simulink model "nms_sim_2D_cost"  (R2024b)
settings: Solver=ode15s  StartTime=0.0  StopTime=t_sim  MaxStep=dt_max  EnableMultiTasking=on
values from neighbouring files (symbols this model uses):
  a_BFSH = param_ctrl(35)*1    [setCtrlPar_optim_CPGreflex2001_2D.m]
  a_GAS = param_ctrl(37)*1    [setCtrlPar_optim_CPGreflex2001_2D.m]
  a_GLU = param_ctrl(31)*1    [setCtrlPar_optim_CPGreflex2001_2D.m]
  a_HAM = param_ctrl(33)*1    [setCtrlPar_optim_CPGreflex2001_2D.m]
  a_HFL = param_ctrl(32)*1    [setCtrlPar_optim_CPGreflex2001_2D.m]
  a_RF = param_ctrl(34)*1    [setCtrlPar_optim_CPGreflex2001_2D.m]
  a_SOL = param_ctrl(38)*1    [setCtrlPar_optim_CPGreflex2001_2D.m]
  a_TA = param_ctrl(39)*1    [setCtrlPar_optim_CPGreflex2001_2D.m]
  a_VAS = param_ctrl(36)*1    [setCtrlPar_optim_CPGreflex2001_2D.m]
  ai = param_ctrl(96)*2.0    [setCtrlPar_optim_CPGreflex2001_2D.m]
  b_BFSH = param_ctrl(52)*.51    [setCtrlPar_optim_CPGreflex2001_2D.m]
  b_BFSHGAS = param_ctrl(55)*.51    [setCtrlPar_optim_CPGreflex2001_2D.m]
  b_BFSHHAM = param_ctrl(54)*.51    [setCtrlPar_optim_CPGreflex2001_2D.m]
  b_BFSHVAS = param_ctrl(53)*.51    [setCtrlPar_optim_CPGreflex2001_2D.m]
  b_GAS = param_ctrl(59)*.51    [setCtrlPar_optim_CPGreflex2001_2D.m]
  b_GASBFSH = param_ctrl(60)*.51    [setCtrlPar_optim_CPGreflex2001_2D.m]
  b_GASSOL = param_ctrl(61)*.51    [setCtrlPar_optim_CPGreflex2001_2D.m]
  b_GLU = param_ctrl(40)*.51    [setCtrlPar_optim_CPGreflex2001_2D.m]
  b_GLUHAM = param_ctrl(42)*.51    [setCtrlPar_optim_CPGreflex2001_2D.m]
  b_GLUHFL = param_ctrl(41)*.51    [setCtrlPar_optim_CPGreflex2001_2D.m]
  b_HAM = param_ctrl(46)*.51    [setCtrlPar_optim_CPGreflex2001_2D.m]
  b_HAMBFSH = param_ctrl(48)*.51    [setCtrlPar_optim_CPGreflex2001_2D.m]
  b_HAMGLU = param_ctrl(47)*.51    [setCtrlPar_optim_CPGreflex2001_2D.m]
  b_HFL = param_ctrl(43)*.51    [setCtrlPar_optim_CPGreflex2001_2D.m]
  b_HFLGLU = param_ctrl(44)*.51    [setCtrlPar_optim_CPGreflex2001_2D.m]
  b_HFLRF = param_ctrl(45)*.51    [setCtrlPar_optim_CPGreflex2001_2D.m]
  b_RF = param_ctrl(49)*.51    [setCtrlPar_optim_CPGreflex2001_2D.m]
  b_RFHFL = param_ctrl(50)*.51    [setCtrlPar_optim_CPGreflex2001_2D.m]
  b_RFVAS = param_ctrl(51)*.51    [setCtrlPar_optim_CPGreflex2001_2D.m]
  b_SOL = param_ctrl(62)*.51    [setCtrlPar_optim_CPGreflex2001_2D.m]
  b_SOLGAS = param_ctrl(64)*.51    [setCtrlPar_optim_CPGreflex2001_2D.m]
  b_SOLTA = param_ctrl(63)*.51    [setCtrlPar_optim_CPGreflex2001_2D.m]
  b_TA = param_ctrl(65)*.51    [setCtrlPar_optim_CPGreflex2001_2D.m]
  b_TASOL = param_ctrl(66)*.51    [setCtrlPar_optim_CPGreflex2001_2D.m]
  b_VAS = param_ctrl(56)*.51    [setCtrlPar_optim_CPGreflex2001_2D.m]
  b_VASBFSH = param_ctrl(57)*.51    [setCtrlPar_optim_CPGreflex2001_2D.m]
  b_VASRF = param_ctrl(58)*.51    [setCtrlPar_optim_CPGreflex2001_2D.m]
  bias = param_ctrl(97)*2.5    [setCtrlPar_optim_CPGreflex2001_2D.m]
  c = 0.05    [nms_MS_2D_scaled.m]
  c_jointstop = 0.3 / (pi/180)    (= 17.1887338539)    [nms_MS_2D_scaled.m]
  D12_F = 0.16    *scaleL_JPhys    [nms_MechInit_2D_scaleSkel.m]
  D12_S = 0.2460	*sub_height    [nms_MechInit_2D_scaleSkel.m]
  D12_T = 0.2450  *sub_height    [nms_MechInit_2D_scaleSkel.m]
  D12y_F = 0.039  *sub_height    [nms_MechInit_2D_scaleSkel.m]
  D12z_HAT = 0.1    [nms_MS_2D_scaled.m]
  D13_F = 0.20    *scaleL_JPhys    [nms_MechInit_2D_scaleSkel.m]
  D1G_F = 0.14    *scaleL_JPhys    [nms_MechInit_2D_scaleSkel.m]
  D1G_HAT = 0.35  *scaleL_JPhys    [nms_MechInit_2D_scaleSkel.m]
  D1G_S = (0.3 - D12y_F/4)	*scaleL_JPhys    [nms_MechInit_2D_scaleSkel.m]
  D1G_T = (0.3 - D12y_F/4)	*scaleL_JPhys    [nms_MechInit_2D_scaleSkel.m]
  D1Gy_F = D12y_F*D1G_F/D12_F    (= 0.07)    [nms_MechInit_2D_scaleSkel.m]
  d_BFSH = param_ctrl(26)*1    [setCtrlPar_optim_CPGreflex2001_2D.m]
  d_GAS = param_ctrl(28)*1    [setCtrlPar_optim_CPGreflex2001_2D.m]
  d_GLU = param_ctrl(22)*1    [setCtrlPar_optim_CPGreflex2001_2D.m]
  d_HAM = param_ctrl(24)*1    [setCtrlPar_optim_CPGreflex2001_2D.m]
  d_HFL = param_ctrl(23)*1    [setCtrlPar_optim_CPGreflex2001_2D.m]
  d_RF = param_ctrl(25)*1    [setCtrlPar_optim_CPGreflex2001_2D.m]
  d_SOL = param_ctrl(29)*1    [setCtrlPar_optim_CPGreflex2001_2D.m]
  d_TA = param_ctrl(30)*1    [setCtrlPar_optim_CPGreflex2001_2D.m]
  d_VAS = param_ctrl(27)*1    [setCtrlPar_optim_CPGreflex2001_2D.m]
  DeltaThRef = 5e-3    (= 0.005)    [nms_MS_2D_scaled.m]
  dloptBFSH = 3.0    (= 3)    [setCtrlPar_optim_CPGreflex2001_2D.m]
  dloptGAS = 3.0    (= 3)    [setCtrlPar_optim_CPGreflex2001_2D.m]
  dloptGLU = 3.0    (= 3)    [setCtrlPar_optim_CPGreflex2001_2D.m]
  dloptHAM = 3.0    (= 3)    [setCtrlPar_optim_CPGreflex2001_2D.m]
  dloptHFL = 3.0    (= 3)    [setCtrlPar_optim_CPGreflex2001_2D.m]
  dloptRF = 3.0    (= 3)    [setCtrlPar_optim_CPGreflex2001_2D.m]
  dloptSOL = 3.0    (= 3)    [setCtrlPar_optim_CPGreflex2001_2D.m]
  dloptTA = 3.0    (= 3)    [setCtrlPar_optim_CPGreflex2001_2D.m]
  dloptVAS = 3.0    (= 3)    [setCtrlPar_optim_CPGreflex2001_2D.m]
  ec_BFSH = param_ctrl(80)*0.15    [setCtrlPar_optim_CPGreflex2001_2D.m]
  ec_GAS = param_ctrl(82)*0.15    [setCtrlPar_optim_CPGreflex2001_2D.m]
  ec_GLU = param_ctrl(76)*0.15    [setCtrlPar_optim_CPGreflex2001_2D.m]
  ec_HAM = param_ctrl(78)*0.15    [setCtrlPar_optim_CPGreflex2001_2D.m]
  ec_HFL = param_ctrl(77)*0.15    [setCtrlPar_optim_CPGreflex2001_2D.m]
  ec_RF = param_ctrl(79)*0.15    [setCtrlPar_optim_CPGreflex2001_2D.m]
  ec_TA = param_ctrl(84)*0.15    [setCtrlPar_optim_CPGreflex2001_2D.m]
  ec_VAS = param_ctrl(81)*0.15    [setCtrlPar_optim_CPGreflex2001_2D.m]
  eref = 0.04    [nms_MS_2D_scaled.m]
  eref_GAS = 0.1    [nms_MS_2D_scaled.m]
  eref_SOL = 0.1    [nms_MS_2D_scaled.m]
  es_BFSH = param_ctrl(89)*0.15    [setCtrlPar_optim_CPGreflex2001_2D.m]
  es_GAS = param_ctrl(91)*0.15    [setCtrlPar_optim_CPGreflex2001_2D.m]
  es_GLU = param_ctrl(85)*0.15    [setCtrlPar_optim_CPGreflex2001_2D.m]
  es_HAM = param_ctrl(87)*0.15    [setCtrlPar_optim_CPGreflex2001_2D.m]
  es_HFL = param_ctrl(86)*0.15    [setCtrlPar_optim_CPGreflex2001_2D.m]
  es_RF = param_ctrl(88)*0.15    [setCtrlPar_optim_CPGreflex2001_2D.m]
  es_TA = param_ctrl(93)*0.15    [setCtrlPar_optim_CPGreflex2001_2D.m]
  es_VAS = param_ctrl(90)*0.15    [setCtrlPar_optim_CPGreflex2001_2D.m]
  FmaxBFSH = 350    [nms_MS_2D_scaled.m]
  FmaxGAS = 2000    [nms_MS_2D_scaled.m]
  FmaxGLU = 4000    [nms_MS_2D_scaled.m]
  FmaxHAM = 2000    [nms_MS_2D_scaled.m]
  FmaxHFL = 2000    [nms_MS_2D_scaled.m]
  FmaxRF = 850    [nms_MS_2D_scaled.m]
  FmaxSOL = 4000    [nms_MS_2D_scaled.m]
  FmaxTA = 800    [nms_MS_2D_scaled.m]
  FmaxVAS = 5000    [nms_MS_2D_scaled.m]
  g = 9.81    [nms_MS_2D_scaled.m]
  gamma_4 = param_ctrl(11) * 1.7    [setCtrlPar_optim_CPGreflexsynergy2023_2D.m]
  h_BFSH = param_ctrl(71)*.1    [setCtrlPar_optim_CPGreflex2001_2D.m]
  h_GAS = param_ctrl(73)*.1    [setCtrlPar_optim_CPGreflex2001_2D.m]
  h_GLU = param_ctrl(67)*.1    [setCtrlPar_optim_CPGreflex2001_2D.m]
  h_HAM = param_ctrl(69)*.1    [setCtrlPar_optim_CPGreflex2001_2D.m]
  h_HFL = param_ctrl(68)*.1    [setCtrlPar_optim_CPGreflex2001_2D.m]
  h_RF = param_ctrl(70)*.1    [setCtrlPar_optim_CPGreflex2001_2D.m]
  h_SOL = param_ctrl(74)*.1    [setCtrlPar_optim_CPGreflex2001_2D.m]
  h_TA = param_ctrl(75)*.1    [setCtrlPar_optim_CPGreflex2001_2D.m]
  h_VAS = param_ctrl(72)*.1    [setCtrlPar_optim_CPGreflex2001_2D.m]
  HLCtrlPar = [theta_tgt l_clr alpha_tgt alpha_cd alpha_cv]    [setCtrlPar_optim_reflex2015_2D.m]
  In_F = 0.005    *scaleM*scaleL_JPhys^2    [nms_MechInit_2D_scaleSkel.m]
  In_HAT = 2.5    *scaleM*scaleL_JPhys^2    [nms_MechInit_2D_scaleSkel.m]
  In_S = 0.05     *scaleM*scaleL_JPhys^2    [nms_MechInit_2D_scaleSkel.m]
  In_T = 0.15     *scaleM*scaleL_JPhys^2    [nms_MechInit_2D_scaleSkel.m]
  init_exc = 0.01    [setInitPar_optim_2D.m]
  init_fm = 0.01    [setInitPar_optim_2D.m]
  init_lce = 1    [setInitPar_optim_2D.m]
  init_LCPG = param_ctrl(12) * 0.01    [setCtrlPar_optim_CPGreflexsynergy2023_2D.m]
  init_LStance = 1    [setInitPar_optim_2D.m]
  init_N1 = osc_signal1(phi_off_osc_ind)    [setCtrlPar_optim_CPGreflex2001_2D.m]
  ... (+441 more)
undefined symbols (not defined in the file or in its folder): cost_act_exponent, cost_v_tgt, flag_controller, Newton, nStep_obj, nStep_startKin, Raphson, sgn, SSW_kin, terrain_slope_angle, v_plateS1, X, Y, Z
libraries: nesl_utility x94, sm_lib x90, simulink x28, simulink_extras x12
(part 18 of 20)

== system nms_sim_2D_cost/Muscle synergy Controller/Right Movement Regulator/Right Trunk Balance ==
  note: GLU
  note: HFL
  theta : Inport
  dtheta : Inport  Port=2
  RStance : EnablePort  StatesWhenEnabling=reset
  Constant : Constant  Value=theta_trunk_tgt
  Constant1 : Constant  Value=k_HFL
  Constant2 : Constant  Value=sigma_HFL
  Constant3 : Constant  Value=theta_trunk_tgt
  Constant4 : Constant  Value=k_GLU
  Constant5 : Constant  Value=sigma_GLU
  Gain : Gain  Gain=-1
  Gain1 : Gain  Gain=-1
  Product{,1..3} (4 alike) : Product
  Sum{,1..3} (4 alike) : Sum  Inputs=|+-
  RExcHFL_MR : Outport  OutputWhenDisabled=reset  InitialOutput=0
  RExcGLU_MR : Outport  Port=2
  wires:
  dtheta/1 -> Product1/2, Product3/2
  Constant3/1 -> Sum2/2
  Constant4/1 -> Gain1/1
  theta/1 -> Sum/1, Sum2/1
  Sum2/1 -> Product2/1  "theta - theta_tgt"
  Gain1/1 -> Product2/2  "-K_GLU"
  Product3/1 -> Sum3/2
  Sum3/1 -> RExcGLU_MR/1
  Product2/1 -> Sum3/1
  Constant5/1 -> Product3/1
  Sum/1 -> Product/1  "theta - theta_tgt"
  Product1/1 -> Sum1/2
  Product/1 -> Sum1/1
  Constant/1 -> Sum/2
  Gain/1 -> Product/2  "-K_HFL"
  Constant2/1 -> Product1/1
  Constant1/1 -> Gain/1
  Sum1/1 -> RExcHFL_MR/1

== system nms_sim_2D_cost/Reflex Controller/Higher Control Layer (Supraspinal Control)/Stance to Swing ==
  LStance : Inport
  RStance : Inport  Port=2
  Lalpha_tgt : Inport  Port=3
  Lphi34 : Inport  Port=4
  Lphi23 : Inport  Port=5
  Ralpha_tgt : Inport  Port=6
  Rphi34 : Inport  Port=7
  Rphi23 : Inport  Port=8
  Abs : Abs  ZeroCross=off  SaturateOnIntegerOverflow=off
  Abs1 : Abs  ZeroCross=off  SaturateOnIntegerOverflow=off
  Lalpha' : Fcn  Expr=u(1) - u(2)/2
  Logical Operator1 : Logic  Operator=NOR  AllPortsSameDT=off  OutDataTypeStr=boolean
  Logical Operator2 : Logic  Operator=NOT  AllPortsSameDT=off
  Logical Operator3 : Logic  AllPortsSameDT=off
  Logical Operator4 : Logic  AllPortsSameDT=off
  Logical Operator5 : Logic  AllPortsSameDT=off
  Mux1 : Mux  Inputs=2
  Mux5 : Mux  Inputs=2
  Ralpha' : Fcn  Expr=u(1) - u(2)/2
  Relational Operator : RelationalOperator  Operator=>  ZeroCross=off  InputSameDT=off
  Sum5 : Sum  Inputs=-+|
  Sum7 : Sum  Inputs=-+|
  LSwInit : Outport  VectorParamsAs1DForOutWhenUnconnected=off
  Flight : Outport  Port=2  VectorParamsAs1DForOutWhenUnconnected=off
  RSwInit : Outport  Port=3  VectorParamsAs1DForOutWhenUnconnected=off
  wires:
  Lalpha'/1 -> Sum7/2  "Lalpha"
  Mux5/1 -> Lalpha'/1
  Ralpha'/1 -> Sum5/2
  Mux1/1 -> Ralpha'/1
  Sum5/1 -> Abs/1
  Sum7/1 -> Abs1/1
  Abs1/1 -> Relational Operator/1
  Abs/1 -> Relational Operator/2
  Logical Operator3/1 -> Logical Operator4/1, Logical Operator5/1
  LStance/1 -> Logical Operator3/1, Logical Operator1/1
  RStance/1 -> Logical Operator3/2, Logical Operator1/2
  Lalpha_tgt/1 -> Sum7/1
  Lphi34/1 -> Mux5/1
  Lphi23/1 -> Mux5/2
  Ralpha_tgt/1 -> Sum5/1
  Rphi34/1 -> Mux1/1
  Rphi23/1 -> Mux1/2
  Logical Operator1/1 -> Flight/1
  Relational Operator/1 -> Logical Operator2/1, Logical Operator4/2
  Logical Operator4/1 -> LSwInit/1
  Logical Operator2/1 -> Logical Operator5/2
  Logical Operator5/1 -> RSwInit/1

== system nms_sim_2D_cost/Reflex Controller/Lower Control Layer (Spinal Cord)/L Stance Phase ==
  note: Left Stance Phase Control
  note: M1: realize compliant leg
  note: M2: prevent knee overextension
  note: M3: balance trunk
  note: 0: Pre-excitations
  note: M5: flex ankle
  note: M4: compensate swing leg
  CtrlPar : Inport
  theta_tgt [rad] : Inport  Port=2
  theta dtheta [rad rad/s] : Inport  Port=3
  CExc_HSw : Inport  Port=4
  FmGLU : Inport  Port=5
  FmHAM : Inport  Port=6
  FmVAS : Inport  Port=7
  LceBFSH : Inport  Port=8
  FmGAS : Inport  Port=9
  FmSOL : Inport  Port=10
  LceTA : Inport  Port=11
  Enable : EnablePort  StatesWhenEnabling=reset  ZeroCross=off
  Demux1 : Demux  Outputs=5
  Demux3 : Demux  Outputs=3
  Demux4 : Demux
  Demux5 : Demux  Outputs=5
  Demux6 : Demux  Outputs=3
  Demux7 : Demux  Outputs=2
  Demux8 : Demux  Outputs=6
  Divide{4..17,19..22,25} (19 alike) : Product
  Gain : Gain  Gain=-1
  Gain2 : Gain  Gain=-1
  Gain3 : Gain  Gain=-1
  Mux{1..3,5} (4 alike) : Mux  Inputs=3
  Mux4 : Mux
  Sum{1,3..5} (4 alike) : Sum  Inputs=-+|  InputSameDT=on  SaturateOnIntegerOverflow=on  OutDataTypeStr=Inherit: Same as first input
  Sum{2,7..8,11} (4 alike) : Sum  Inputs=|++  InputSameDT=on  SaturateOnIntegerOverflow=on  OutDataTypeStr=Inherit: Same as first input
  Sum6 : Sum  Inputs=+-|  InputSameDT=on  SaturateOnIntegerOverflow=on  OutDataTypeStr=Inherit: Same as first input
  parStPreE : Selector  InputPortWidth=St_i  IndexOptions=Index vector (dialog)  Indices=parSt_PreE_i  OutputSizes=1
  parSt_M1 : Selector  InputPortWidth=St_i  IndexOptions=Index vector (dialog)  Indices=parSt_M1_i  OutputSizes=1
  parSt_M2 : Selector  InputPortWidth=St_i  IndexOptions=Index vector (dialog)  Indices=parSt_M2_i  OutputSizes=1
  parSt_M3 : Selector  InputPortWidth=St_i  IndexOptions=Index vector (dialog)  Indices=parSt_M3_i  OutputSizes=1
  parSt_M4 : Selector  InputPortWidth=St_i  IndexOptions=Index vector (dialog)  Indices=parSt_M4_i  OutputSizes=1
  parSt_M5 : Selector  InputPortWidth=St_i  IndexOptions=Index vector (dialog)  Indices=parSt_M5_i  OutputSizes=1
  positive half{1..6} (6 alike) : Saturate  UpperLimit=inf  LowerLimit=0  ZeroCross=off
  E_St_0 : Outport  OutputWhenDisabled=reset  InitialOutput=0  VectorParamsAs1DForOutWhenUnconnected=off
  E_M1 [GLU VAS SOL] : Outport  Port=2  OutputWhenDisabled=reset  InitialOutput=0  VectorParamsAs1DForOutWhenUnconnected=off
  E_M2 [HAM VAS BFSH GAS] : Outport  Port=3  OutputWhenDisabled=reset  InitialOutput=0  VectorParamsAs1DForOutWhenUnconnected=off
  E_M3 [HFL GLU HAM] : Outport  Port=4  OutputWhenDisabled=reset  InitialOutput=0  VectorParamsAs1DForOutWhenUnconnected=off
  E_M4 [HFL GLU HAM] : Outport  Port=5  OutputWhenDisabled=reset  InitialOutput=0  VectorParamsAs1DForOutWhenUnconnected=off
  E_M5 [TA] : Outport  Port=6  OutputWhenDisabled=reset  InitialOutput=0  VectorParamsAs1DForOutWhenUnconnected=off
  wires:
  Demux5/2 -> Divide20/2  "GainDTh_HFL"
  Divide11/1 -> Mux4/4  "GAS"
  Divide15/1 -> Gain/1
  Divide13/1 -> Mux4/3  "BFSH"
  Mux2/1 -> E_M1 [GLU VAS SOL]/1
  positive half3/1 -> Divide15/1
  Demux8/2 -> Sum3/1  "loff_BFSH_VAS"
  Demux8/6 -> Divide11/1  "FGain_GAS"
  Demux8/5 -> Divide13/2  "LGain_BFSH"
  Sum3/1 -> positive half3/1
  Divide7/1 -> Mux2/1  "GLU"
  LceBFSH/1 -> Sum3/2, Sum4/2
  Demux5/1 -> Divide19/2  "GainTh_HFL"
  FmGLU/1 -> Divide7/2
  parSt_M1/1 -> Demux3/1
  positive half6/1 -> Mux1/3
  Demux7/2 -> Gain3/1, Divide5/1  "dtheta"
  Sum2/1 -> positive half1/1  "HFL"
  Sum4/1 -> positive half4/1
  Divide10/1 -> Mux2/3  "SOL"
  positive half2/1 -> Mux1/2
  Divide14/1 -> Mux4/1  "HAM"
  theta_tgt [rad]/1 -> Sum1/1
  Demux5/5 -> Divide6/2  "SGainGLU_HAM"
  Divide6/1 -> positive half6/1  "HAM"
  positive half1/1 -> Mux1/1
  Mux1/1 -> E_M3 [HFL GLU HAM]/1
  Divide5/1 -> Sum8/2
  Demux8/3 -> Divide15/2  "LGainBFSH_VAS"
  parSt_M2/1 -> Demux8/1
  Demux8/1 -> Divide14/1  "FGain_HAM"
  Gain/1 -> Mux4/2  "VAS"
  Sum8/1 -> Divide6/1, positive half2/1  "GLU"
  Demux5/3 -> Divide4/2  "GainTh_GLU"
  Gain2/1 -> Divide19/1
  Divide20/1 -> Sum2/2
  Gain3/1 -> Divide20/1
  Divide19/1 -> Sum2/1
  parSt_M3/1 -> Demux5/1
  Divide4/1 -> Sum8/1
  Demux3/3 -> Divide10/1  "FGain_SOL"
  FmHAM/1 -> Divide14/2
  theta dtheta [rad rad/s]/1 -> Demux7/1
  Sum1/1 -> Gain2/1, Divide4/1
  Demux7/1 -> Sum1/2  "theta"
  Demux5/4 -> Divide5/2  "GainDTh_GLU"
  FmGAS/1 -> Divide11/2
  Demux8/4 -> Sum4/1  "loff_BFSH"
  FmVAS/1 -> Divide8/2
  Demux3/1 -> Divide7/1  "FGain_GLU"
  positive half4/1 -> Divide13/1
  Divide8/1 -> Mux2/2  "VAS"
  Demux3/2 -> Divide8/1  "FGain_VAS"
  Mux4/1 -> E_M2 [HAM VAS BFSH GAS]/1
  parStPreE/1 -> E_St_0/1
  Sum6/1 -> E_M5 [TA]/1  "TA"
  Demux1/5 -> Divide21/2  "SGainGLU_HAM"
  Divide12/1 -> Sum11/1
  Sum11/1 -> Mux5/2, Divide21/1  "GLU"
  Demux4/4 -> Divide9/2  "Exc_CRF"
  Divide21/1 -> Mux5/3  "HAM"
  CExc_HSw/1 -> Demux4/1
  Demux1/4 -> Divide9/1  "SGainCRF_GLU"
  Divide17/1 -> Sum7/2
  Demux1/2 -> Divide17/1  "SGainCHAM_HFL"
  Demux4/2 -> Divide22/2  "Exc_CGLU"
  Sum7/1 -> Mux5/1  "HFL"
  positive half5/1 -> Divide16/1
  Demux1/1 -> Divide22/1  "SGainCGLU_HFL"
  Demux4/1 -> Divide12/2  "Exc_CHFL"
  Demux4/3 -> Divide17/2  "Exc_CHAM"
  Divide9/1 -> Sum11/2
  Demux1/3 -> Divide12/1  "SGainCHFL_GLU"
  parSt_M4/1 -> Demux1/1
  Demux6/3 -> Divide25/2  "FGainSOL_TA"
  Demux6/1 -> Sum5/1  "loffTA"
  Demux6/2 -> Divide16/2  "LGain_TA"
  CtrlPar/1 -> parStPreE/1, parSt_M1/1, parSt_M2/1, parSt_M5/1, parSt_M4/1, parSt_M3/1
  Divide25/1 -> Sum6/2
  Mux5/1 -> E_M4 [HFL GLU HAM]/1
  Divide22/1 -> Sum7/1
  Sum5/1 -> positive half5/1
  Divide16/1 -> Sum6/1
  parSt_M5/1 -> Demux6/1
  FmSOL/1 -> Divide25/1, Divide10/2
  LceTA/1 -> Sum5/2

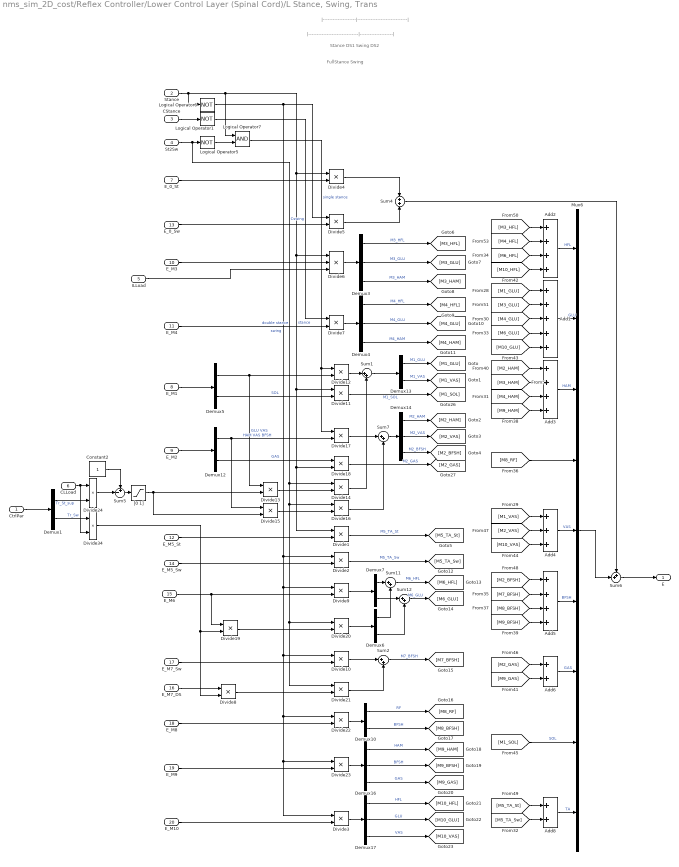
== system nms_sim_2D_cost/Reflex Controller/Lower Control Layer (Spinal Cord)/L Stance, Swing, Trans ==
  note: Stance DS1 Swing DS2
  note: FullStance Swing
  note: |------------------------------|--------------------|
  note: |--------------------|------------------------------|
  CtrlPar : Inport
  Stance : Inport  Port=2
  CStance : Inport  Port=3
  St2Sw : Inport  Port=4
  ILLoad : Inport  Port=5
  CLLoad : Inport  Port=6
  E_0_St : Inport  Port=7
  E_M1 : Inport  Port=8
  E_M2 : Inport  Port=9
  E_M3 : Inport  Port=10
  E_M4 : Inport  Port=11
  E_M5_St : Inport  Port=12
  E_0_Sw : Inport  Port=13
  E_M5_Sw : Inport  Port=14
  E_M6 : Inport  Port=15
  E_M7_DS : Inport  Port=16
  E_M7_Sw : Inport  Port=17
  E_M8 : Inport  Port=18
  E_M9 : Inport  Port=19
  E_M10 : Inport  Port=20
  Add1 : Sum  Inputs=5
  Add2 : Sum  Inputs=4
  Add3 : Sum  Inputs=4
  Add4 : Sum  Inputs=3
  Add5 : Sum  Inputs=4
  Add6 : Sum  Inputs=2
  Add8 : Sum  Inputs=2
  Constant2 : Constant
  Demux{1,6..7,10,13} (5 alike) : Demux  Outputs=2
  Demux12 : Demux  Outputs=[3 1]
  Demux{3..4,14,16..17} (5 alike) : Demux  Outputs=3
  Demux5 : Demux  Outputs=[2 1]
  Divide{1..5,7..24,34} (24 alike) : Product
  Divide6 : Product  Inputs=3
  Logical Operator1 : Logic  Operator=NOT  AllPortsSameDT=off  OutDataTypeStr=boolean
  Logical Operator5 : Logic  Operator=NOT  AllPortsSameDT=off  OutDataTypeStr=boolean
  Logical Operator6 : Logic  Operator=NOT  AllPortsSameDT=off  OutDataTypeStr=boolean
  Logical Operator7 : Logic  AllPortsSameDT=off  OutDataTypeStr=boolean
  Mux6 : Mux  Inputs=9
  Sum{1..2,7,11..12} (5 alike) : Sum  Inputs=|++  InputSameDT=on  SaturateOnIntegerOverflow=on  OutDataTypeStr=Inherit: Same as first input
  Sum4 : Sum  InputSameDT=on  SaturateOnIntegerOverflow=on  OutDataTypeStr=Inherit: Same as first input
  Sum5 : Sum  Inputs=+-|  InputSameDT=on  SaturateOnIntegerOverflow=on  OutDataTypeStr=Inherit: Same as first input
  Sum6 : Sum  Inputs=++|  InputSameDT=on  SaturateOnIntegerOverflow=on  OutDataTypeStr=Inherit: Same as first input
  "[0 1]" : Saturate  UpperLimit=1  LowerLimit=0  ZeroCross=off
  E : Outport  OutputWhenDisabled=reset  InitialOutput=0  VectorParamsAs1DForOutWhenUnconnected=off
  wires:
  CtrlPar/1 -> Demux1/1
  Stance/1 -> Logical Operator6/1, Logical Operator7/1, Divide4/1, Divide11/1, Divide18/2, Divide1/1, Divide6/1  "stance"
  St2Sw/1 -> Logical Operator5/1, Divide14/1, Divide16/1, Divide20/1, Divide21/1  "double stance"
  Logical Operator5/1 -> Logical Operator7/2
  E_M4/1 -> Divide7/2
  CStance/1 -> Logical Operator1/1
  Logical Operator1/1 -> Divide7/1  "Cswing"
  Demux1/1 -> Divide24/2  "Tr_St_sup"
  Divide24/1 -> Sum5/2
  Constant2/1 -> Sum5/1
  CLLoad/1 -> Divide24/1, Divide34/2
  Demux4/1 -> [M4_HFL]  "M4_HFL"
  Add2/1 -> Mux6/1  "HFL"
  Add1/1 -> Mux6/2  "GLU"
  Demux4/2 -> [M4_GLU]  "M4_GLU"
  Add3/1 -> Mux6/3  "HAM"
  Demux4/3 -> [M4_HAM]  "M4_HAM"
  Add4/1 -> Mux6/5  "VAS"
  Add5/1 -> Mux6/6  "BFSH"
  Add6/1 -> Mux6/7  "GAS"
  Add8/1 -> Mux6/9  "TA"
  Demux1/2 -> Divide34/1  "Tr_Sw"
  Divide7/1 -> Demux4/1
  Logical Operator7/1 -> Divide12/1, Divide17/1  "single stance"
  Divide34/1 -> Divide19/2, Divide8/2
  Logical Operator6/1 -> Divide5/1, Divide2/1, Divide9/1, Divide10/1, Divide23/1, Divide3/1, Divide22/1  "swing"
  Mux6/1 -> Sum6/2
  Sum6/1 -> E/1
  Sum4/1 -> Sum6/1
  E_0_Sw/1 -> Divide5/2
  E_0_St/1 -> Divide4/2
  Divide5/1 -> Sum4/2
  Divide4/1 -> Sum4/1
  E_M1/1 -> Demux5/1
  E_M2/1 -> Demux12/1
  Demux5/1 -> Divide12/2, Divide13/1  "GLU VAS"
  Demux5/2 -> Divide11/2  "SOL"
  Divide12/1 -> Sum1/1
  Divide13/1 -> Divide14/2
  Divide14/1 -> Sum1/2
  Divide16/1 -> Sum7/2
  Divide15/1 -> Divide16/2
  Sum1/1 -> Demux13/1
  Demux13/1 -> [M1_GLU]  "M1_GLU"
  Demux13/2 -> [M1_VAS]  "M1_VAS"
  Demux12/1 -> Divide17/2, Divide15/1  "HAM VAS BFSH"
  Divide17/1 -> Sum7/1
  Sum7/1 -> Demux14/1
  Demux14/1 -> [M2_HAM]  "M2_HAM"
  Demux14/2 -> [M2_VAS]  "M2_VAS"
  Demux14/3 -> [M2_BFSH]  "M2_BFSH"
  Demux12/2 -> Divide18/1  "GAS"
  Divide18/1 -> [M2_GAS]  "M2_GAS"
  E_M5_St/1 -> Divide1/2
  Divide1/1 -> [M5_TA_St]  "M5_TA_St"
  Divide11/1 -> [M1_SOL]  "M1_SOL"
  E_M3/1 -> Divide6/2
  ILLoad/1 -> Divide6/3
  Divide6/1 -> Demux3/1
  Demux3/1 -> [M3_HFL]  "M3_HFL"
  Demux3/2 -> [M3_GLU]  "M3_GLU"
  Demux3/3 -> [M3_HAM]  "M3_HAM"
  E_M5_Sw/1 -> Divide2/2
  Divide2/1 -> [M5_TA_Sw]  "M5_TA_Sw"
  E_M6/1 -> Divide9/2, Divide19/1
  Divide9/1 -> Demux7/1
  Demux7/2 -> Sum12/1
  Divide20/1 -> Demux6/1
  Demux6/1 -> Sum11/2
  Demux6/2 -> Sum12/2
  Demux7/1 -> Sum11/1
  Divide19/1 -> Divide20/2
  Sum11/1 -> [M6_HFL]  "M6_HFL"
  Sum12/1 -> [M6_GLU]  "M6_GLU"
  Divide10/1 -> Sum2/1
  Divide21/1 -> Sum2/2
  Sum5/1 -> "[0 1]"/1
  E_M7_Sw/1 -> Divide10/2
  Divide8/1 -> Divide21/2
  E_M7_DS/1 -> Divide8/1
  Sum2/1 -> [M7_BFSH]  "M7_BFSH"
  E_M8/1 -> Divide22/2
  Divide22/1 -> Demux10/1
  E_M9/1 -> Divide23/2
  Divide23/1 -> Demux16/1
  E_M10/1 -> Divide3/2
  Divide3/1 -> Demux17/1
  Demux10/2 -> [M8_BFSH]  "BFSH"
  Demux10/1 -> [M8_RF]  "RF"
  Demux16/1 -> [M9_HAM]  "HAM"
  Demux16/2 -> [M9_BFSH]  "BFSH"
  Demux16/3 -> [M9_GAS]  "GAS"
  Demux17/1 -> [M10_HFL]  "HFL"
  Demux17/2 -> [M10_GLU]  "GLU"
  Demux17/3 -> [M10_VAS]  "VAS"
  [M1_GLU] -> Add1/1
  [M3_GLU] -> Add1/2
  [M4_GLU] -> Add1/3
  [M6_GLU] -> Add1/4
  [M10_GLU] -> Add1/5
  [M1_VAS] -> Add4/1
  [M2_HAM] -> Add3/1
  [M2_VAS] -> Add4/2
  [M2_BFSH] -> Add5/1
  [M2_GAS] -> Add6/1
  [M3_HFL] -> Add2/1
  [M3_HAM] -> Add3/2
  [M4_HFL] -> Add2/2
  [M4_HAM] -> Add3/3
  [M5_TA_St] -> Add8/1
  [M5_TA_Sw] -> Add8/2
  [M6_HFL] -> Add2/3
  [M7_BFSH] -> Add5/2
  [M9_BFSH] -> Add5/4
  [M8_BFSH] -> Add5/3
  [M8_RF] -> Mux6/4
  [M9_HAM] -> Add3/4
  [M9_GAS] -> Add6/2
  [M10_HFL] -> Add2/4
  [M10_VAS] -> Add4/3
  [M1_SOL] -> Mux6/8  "SOL"
  "[0 1]"/1 -> Divide15/2, Divide13/2

== system nms_sim_2D_cost/Reflex Controller/Lower Control Layer (Spinal Cord)/L Swing Phase ==
  note: Left Swing Phase Control
  note: 0: Pre-excitations
  note: M6: swing hip
  note: M7: flex knee
  note: M8: hold knee
  note: M9: stop leg
  note: M10: prepare stance
  note: M5: flex ankle
  CtrlPar : Inport
  Stance : Inport  Port=2
  a_tgt : Inport  Port=3
  l_clr : Inport  Port=4
  LceRF : Inport  Port=5
  VceRF : Inport  Port=6
  LceHAM : Inport  Port=7
  VceHAM : Inport  Port=8
  lceBFSH : Inport  Port=9
  VceVAS : Inport  Port=10
  VceBFSH : Inport  Port=11
  LceHFL : Inport  Port=12
  LceGLU : Inport  Port=13
  LceVAS : Inport  Port=14
  LceTA : Inport  Port=15
  Enable : EnablePort  StatesWhenEnabling=reset  ZeroCross=off
  Constant1 : Constant  Value=0  OutDataTypeStr=boolean
  Constant10 : Constant  Value=leg_l
  Constant2 : Constant
  Constant3 : Constant
  Constant5 : Constant
  Demux1 : Demux  Outputs=2
  Demux2 : Demux  Outputs=2
  Demux4 : Demux  Outputs=9
  Divide{1..8,22} (9 alike) : Product
  Gain1 : Gain  Gain=-1
  Logical Operator : Logic  Operator=NOT  AllPortsSameDT=off  OutDataTypeStr=boolean
  Logical Operator1 : Logic  AllPortsSameDT=off  OutDataTypeStr=boolean
  Logical Operator2 : Logic  Operator=NOT  AllPortsSameDT=off  OutDataTypeStr=boolean
  Mux1 : Mux  Inputs=3
  Mux2 : Mux  Inputs=2
  Mux3 : Mux  Inputs=2
  Mux4 : Mux  Inputs=3
  Mux8 : Mux  Inputs=2
  Relational Operator : RelationalOperator  Operator=<=  OutDataTypeStr=boolean  ZeroCross=off  InputSameDT=off
  S-R Flip-Flop : simulink_extras/Flip Flops/S-R Flip-Flop  initial_condition=0
  Sum1 : Sum  Inputs=-+|  InputSameDT=on  SaturateOnIntegerOverflow=on  OutDataTypeStr=Inherit: Same as first input
  Sum10 : Sum  Inputs=++|  InputSameDT=on  SaturateOnIntegerOverflow=on  OutDataTypeStr=Inherit: Same as first input
  Sum13 : Sum  Inputs=|+-  InputSameDT=on  SaturateOnIntegerOverflow=on  OutDataTypeStr=Inherit: Same as first input
  Sum14 : Sum  Inputs=|+-  InputSameDT=on  SaturateOnIntegerOverflow=on  OutDataTypeStr=Inherit: Same as first input
  Sum2 : Sum  Inputs=++|  InputSameDT=on  SaturateOnIntegerOverflow=on  OutDataTypeStr=Inherit: Same as first input
  Sum3 : Sum  Inputs=-+|  InputSameDT=on  SaturateOnIntegerOverflow=on  OutDataTypeStr=Inherit: Same as first input
  Sum4 : Sum  Inputs=|+-  InputSameDT=on  SaturateOnIntegerOverflow=on  OutDataTypeStr=Inherit: Same as first input
  Sum5 : Sum  Inputs=+-|  InputSameDT=on  SaturateOnIntegerOverflow=on  OutDataTypeStr=Inherit: Same as first input
  Sum6 : Sum  Inputs=|++  InputSameDT=on  SaturateOnIntegerOverflow=on  OutDataTypeStr=Inherit: Same as first input
  Sum7 : Sum  Inputs=|++  InputSameDT=on  SaturateOnIntegerOverflow=on  OutDataTypeStr=Inherit: Same as first input
  Sum8 : Sum  Inputs=++|  InputSameDT=on  SaturateOnIntegerOverflow=on  OutDataTypeStr=Inherit: Same as first input
  Sum9 : Sum  Inputs=+-|  InputSameDT=on  SaturateOnIntegerOverflow=on  OutDataTypeStr=Inherit: Same as first input
  Terminator : Terminator
  kneei_flexion from alpha : Subsystem  TreatAsAtomicUnit=on
  kneeii_damp and hold & kneeiii_leg stop & kneeiv_stance preparation : Subsystem  TreatAsAtomicUnit=on
  negative half : Saturate  UpperLimit=0  LowerLimit=-inf  ZeroCross=off
  negative half1 : Saturate  UpperLimit=0  LowerLimit=-inf  ZeroCross=off
  negative half2 : Saturate  UpperLimit=0  LowerLimit=-inf  ZeroCross=off
  parSwA : Selector  InputPortWidth=Sw_i  IndexOptions=Index vector (dialog)  Indices=parSwA_i  OutputSizes=1
  parSwH : Selector  InputPortWidth=Sw_i  IndexOptions=Index vector (dialog)  Indices=parSwH_i  OutputSizes=1
  parSwKi : Selector  InputPortWidth=Sw_i  IndexOptions=Index vector (dialog)  Indices=parSwKi_i  OutputSizes=1
  parSwPhi : Selector  InputPortWidth=Sw_i  IndexOptions=Index vector (dialog)  Indices=parSwPhi_i  OutputSizes=1
  parSwPreE : Selector  InputPortWidth=Sw_i  IndexOptions=Index vector (dialog)  Indices=parSwPreE_i  OutputSizes=1
  phi_clr : Fcn  Expr=acos((u(2)^2+u(3)^2-u(1)^2)/(2*u(2)*u(3)))
  positive half1 : Saturate  UpperLimit=inf  LowerLimit=0  ZeroCross=off
  positive half2 : Saturate  UpperLimit=inf  LowerLimit=0  ZeroCross=off
  positive half3 : Saturate  UpperLimit=inf  LowerLimit=0  ZeroCross=off
  E_Sw_0 : Outport  OutputWhenDisabled=reset  InitialOutput=0  VectorParamsAs1DForOutWhenUnconnected=off
  E_M5_Sw [TA] : Outport  Port=2  OutputWhenDisabled=reset  InitialOutput=0  VectorParamsAs1DForOutWhenUnconnected=off
  E_M6 [HFL GLU] : Outport  Port=3  OutputWhenDisabled=reset  InitialOutput=0  VectorParamsAs1DForOutWhenUnconnected=off
  E_M7_DS [BFSH] : Outport  Port=4  OutputWhenDisabled=reset  InitialOutput=0  VectorParamsAs1DForOutWhenUnconnected=off
  E_M7_Sw [BFSH] : Outport  Port=5  OutputWhenDisabled=reset  InitialOutput=0  VectorParamsAs1DForOutWhenUnconnected=off
  M8 [RF BFSH] : Outport  Port=6  OutputWhenDisabled=reset  InitialOutput=0  VectorParamsAs1DForOutWhenUnconnected=off
  M9 [HAM BFSH GAS] : Outport  Port=7  OutputWhenDisabled=reset  InitialOutput=0  VectorParamsAs1DForOutWhenUnconnected=off
  M10 [HFL GLU VAS] : Outport  Port=8  OutputWhenDisabled=reset  InitialOutput=0  VectorParamsAs1DForOutWhenUnconnected=off
  wires:
  CtrlPar/1 -> parSwA/1, parSwPreE/1, parSwH/1, kneeii_damp and hold & kneeiii_leg stop & kneeiv_stance preparation/1(CtrlPar), parSwPhi/1, parSwKi/1
  parSwH/1 -> Demux4/1
  Constant5/1 -> Sum10/1
  a_tgt/1 -> Sum2/1, kneeii_damp and hold & kneeiii_leg stop & kneeiv_stance preparation/2(a_tgt), Sum13/1
  Demux4/2 -> Sum13/2  "aRef_RF"
  Sum13/1 -> Divide22/2
  Demux4/1 -> Divide22/1  "a2lopt_RF"
  Divide22/1 -> Sum10/2
  Sum10/1 -> Sum1/1  "lceOffRF"
  Sum1/1 -> positive half2/1  "del_LceRF"
  positive half2/1 -> Divide5/1  "del_lce"
  Demux4/3 -> Divide5/2  "LGainRF_HFL"
  Demux4/6 -> Sum2/2  "a_del"
  Sum2/1 -> Sum4/1  "a_thr"
  Demux4/7 -> Sum4/2  "aRef_HAM"
  Sum4/1 -> Divide1/2
  Demux4/5 -> Divide1/1  "a2lopt_HAM"
  Constant2/1 -> Sum5/1
  Divide1/1 -> Sum5/2
  Sum3/1 -> positive half1/1
  positive half1/1 -> Divide2/1
  Demux4/8 -> Divide2/2  "LGainHAM_GLU"
  Sum5/1 -> Sum3/1  "lceOffHAM"
  LceHAM/1 -> Sum3/2, kneeii_damp and hold & kneeiii_leg stop & kneeiv_stance preparation/4(LceHAM)
  Gain1/1 -> Divide3/1
  negative half/1 -> Gain1/1  "-VceRF"
  parSwKi/1 -> Divide3/2  "VGainRF_BFSH"
  Divide3/1 -> kneei_flexion from alpha/1(SBFSH), E_M7_DS [BFSH]/1  "BFSH"
  Constant1/1 -> S-R Flip-Flop/2
  S-R Flip-Flop/2 -> Terminator/1
  S-R Flip-Flop/1 -> Logical Operator/1, kneeii_damp and hold & kneeiii_leg stop & kneeiv_stance preparation/Enable
  Logical Operator/1 -> kneei_flexion from alpha/Enable
  lceBFSH/1 -> Relational Operator/1
  Mux8/1 -> phi_clr/1
  l_clr/1 -> Mux8/1
  Constant10/1 -> Mux8/2
  parSwPhi/1 -> Demux1/1
  Sum9/1 -> Divide4/2
  Demux1/1 -> Divide4/1  "phi2lopt_BFSH"
  Demux1/2 -> Sum9/2  "phiRef_BFSH"
  phi_clr/1 -> Sum9/1
  Constant3/1 -> Sum8/1
  Divide4/1 -> Sum8/2
  Sum8/1 -> Relational Operator/2  "lceOffLClr_BFSH"
  VceBFSH/1 -> kneeii_damp and hold & kneeiii_leg stop & kneeiv_stance preparation/7(VceBFSH)
  LceHFL/1 -> kneeii_damp and hold & kneeiii_leg stop & kneeiv_stance preparation/9(LceHFL)  "LceHFL"
  LceGLU/1 -> kneeii_damp and hold & kneeiii_leg stop & kneeiv_stance preparation/10(LceGLU)
  LceVAS/1 -> kneeii_damp and hold & kneeiii_leg stop & kneeiv_stance preparation/11(LceVAS)
  kneeii_damp and hold & kneeiii_leg stop & kneeiv_stance preparation/6(SHFL_Sw_kiv) -> Mux1/1
  kneeii_damp and hold & kneeiii_leg stop & kneeiv_stance preparation/7(SGLU_Sw_kiv) -> Mux1/2
  kneei_flexion from alpha/1(SBFSH_Sw_ki) -> E_M7_Sw [BFSH]/1
  kneeii_damp and hold & kneeiii_leg stop & kneeiv_stance preparation/2(SBFSH_Sw_kii) -> Mux3/2
  kneeii_damp and hold & kneeiii_leg stop & kneeiv_stance preparation/4(SBFSH_Sw_kiii) -> Mux4/2
  parSwA/1 -> Demux2/1
  Demux2/1 -> Divide6/1  "LGainTA"
  Sum14/1 -> positive half3/1
  LceTA/1 -> Sum14/1
  positive half3/1 -> Divide6/2
  Demux2/2 -> Sum14/2  "LceOffTA"
  Logical Operator1/1 -> S-R Flip-Flop/1
  Relational Operator/1 -> Logical Operator1/2
  Stance/1 -> Logical Operator2/1
  Logical Operator2/1 -> Logical Operator1/1
  parSwPreE/1 -> E_Sw_0/1
  kneeii_damp and hold & kneeiii_leg stop & kneeiv_stance preparation/3(SHAM_Sw_kiii) -> Mux4/1  "HAM"
  kneeii_damp and hold & kneeiii_leg stop & kneeiv_stance preparation/1(SRF_Sw_kii) -> Mux3/1  "RF"
  kneeii_damp and hold & kneeiii_leg stop & kneeiv_stance preparation/8(SVAS_Sw_kiv) -> Mux1/3  "VAS"
  Divide6/1 -> E_M5_Sw [TA]/1  "TA"
  kneeii_damp and hold & kneeiii_leg stop & kneeiv_stance preparation/5(SGAS_Sw_kiii) -> Mux4/3  "GAS"
  Mux2/1 -> E_M6 [HFL GLU]/1
  Mux3/1 -> M8 [RF BFSH]/1
  Mux4/1 -> M9 [HAM BFSH GAS]/1
  Mux1/1 -> M10 [HFL GLU VAS]/1
  LceRF/1 -> Sum1/2, kneeii_damp and hold & kneeiii_leg stop & kneeiv_stance preparation/3(LceRF)  "LceRF"
  VceVAS/1 -> kneeii_damp and hold & kneeiii_leg stop & kneeiv_stance preparation/6(VceVAS)
  Demux4/4 -> Divide7/1  "Sw_VGainRF_HFL"
  Demux4/9 -> Divide8/1  "Sw_VGainHAM_GLU"
  VceRF/1 -> negative half1/1, kneeii_damp and hold & kneeiii_leg stop & kneeiv_stance preparation/8(VceRF), negative half/1  "VceRF"
  VceHAM/1 -> kneeii_damp and hold & kneeiii_leg stop & kneeiv_stance preparation/5(VceHAM), negative half2/1
  Divide5/1 -> Sum6/1  "HFL"
  Divide7/1 -> Sum6/2
  Sum6/1 -> Mux2/1  "HFL"
  negative half1/1 -> Divide7/2
  negative half2/1 -> Divide8/2
  Divide2/1 -> Sum7/1  "GLU"
  Sum7/1 -> Mux2/2  "GLU"
  Divide8/1 -> Sum7/2

== system nms_sim_2D_cost/Reflex Controller/Lower Control Layer (Spinal Cord)/R Stance Phase ==
  note: Left Stance Phase Control
  note: M1: realize compliant leg
  note: M2: prevent knee overextension
  note: M3: balance trunk
  note: 0: Pre-excitations
  note: M5: flex ankle
  note: M4: compensate swing leg
  CtrlPar : Inport
  theta_tgt [rad] : Inport  Port=2
  theta dtheta [rad rad/s] : Inport  Port=3
  CExc_HSw : Inport  Port=4
  FmGLU : Inport  Port=5
  FmHAM : Inport  Port=6
  FmVAS : Inport  Port=7
  LceBFSH : Inport  Port=8
  FmGAS : Inport  Port=9
  FmSOL : Inport  Port=10
  LceTA : Inport  Port=11
  Enable : EnablePort  StatesWhenEnabling=reset  ZeroCross=off
  Demux1 : Demux  Outputs=5
  Demux3 : Demux  Outputs=3
  Demux4 : Demux
  Demux5 : Demux  Outputs=5
  Demux6 : Demux  Outputs=3
  Demux7 : Demux  Outputs=2
  Demux8 : Demux  Outputs=6
  Divide{4..17,19..22,25} (19 alike) : Product
  Gain : Gain  Gain=-1
  Gain2 : Gain  Gain=-1
  Gain3 : Gain  Gain=-1
  Mux{1..3,5} (4 alike) : Mux  Inputs=3
  Mux4 : Mux
  Sum{1,3..5} (4 alike) : Sum  Inputs=-+|  InputSameDT=on  SaturateOnIntegerOverflow=on  OutDataTypeStr=Inherit: Same as first input
  Sum{2,7..8,11} (4 alike) : Sum  Inputs=|++  InputSameDT=on  SaturateOnIntegerOverflow=on  OutDataTypeStr=Inherit: Same as first input
  Sum6 : Sum  Inputs=+-|  InputSameDT=on  SaturateOnIntegerOverflow=on  OutDataTypeStr=Inherit: Same as first input
  parStPreE : Selector  InputPortWidth=St_i  IndexOptions=Index vector (dialog)  Indices=parSt_PreE_i  OutputSizes=1
  parSt_M1 : Selector  InputPortWidth=St_i  IndexOptions=Index vector (dialog)  Indices=parSt_M1_i  OutputSizes=1
  parSt_M2 : Selector  InputPortWidth=St_i  IndexOptions=Index vector (dialog)  Indices=parSt_M2_i  OutputSizes=1
  parSt_M3 : Selector  InputPortWidth=St_i  IndexOptions=Index vector (dialog)  Indices=parSt_M3_i  OutputSizes=1
  parSt_M4 : Selector  InputPortWidth=St_i  IndexOptions=Index vector (dialog)  Indices=parSt_M4_i  OutputSizes=1
  parSt_M5 : Selector  InputPortWidth=St_i  IndexOptions=Index vector (dialog)  Indices=parSt_M5_i  OutputSizes=1
  positive half{1..6} (6 alike) : Saturate  UpperLimit=inf  LowerLimit=0  ZeroCross=off
  E_St_0 : Outport  OutputWhenDisabled=reset  InitialOutput=0  VectorParamsAs1DForOutWhenUnconnected=off
  E_M1 [GLU VAS SOL] : Outport  Port=2  OutputWhenDisabled=reset  InitialOutput=0  VectorParamsAs1DForOutWhenUnconnected=off
  E_M2 [HAM VAS BFSH GAS] : Outport  Port=3  OutputWhenDisabled=reset  InitialOutput=0  VectorParamsAs1DForOutWhenUnconnected=off
  E_M3 [HFL GLU HAM] : Outport  Port=4  OutputWhenDisabled=reset  InitialOutput=0  VectorParamsAs1DForOutWhenUnconnected=off
  E_M4 [HFL GLU HAM] : Outport  Port=5  OutputWhenDisabled=reset  InitialOutput=0  VectorParamsAs1DForOutWhenUnconnected=off
  E_M5 [TA] : Outport  Port=6  OutputWhenDisabled=reset  InitialOutput=0  VectorParamsAs1DForOutWhenUnconnected=off
  wires:
  Demux5/2 -> Divide20/2  "GainDTh_HFL"
  Divide11/1 -> Mux4/4  "GAS"
  Divide15/1 -> Gain/1
  Divide13/1 -> Mux4/3  "BFSH"
  Mux2/1 -> E_M1 [GLU VAS SOL]/1
  positive half3/1 -> Divide15/1
  Demux8/2 -> Sum3/1  "loff_BFSH_VAS"
  Demux8/6 -> Divide11/1  "FGain_GAS"
  Demux8/5 -> Divide13/2  "LGain_BFSH"
  Sum3/1 -> positive half3/1
  Divide7/1 -> Mux2/1  "GLU"
  LceBFSH/1 -> Sum3/2, Sum4/2
  Demux5/1 -> Divide19/2  "GainTh_HFL"
  FmGLU/1 -> Divide7/2
  parSt_M1/1 -> Demux3/1
  positive half6/1 -> Mux1/3
  Demux7/2 -> Gain3/1, Divide5/1  "dtheta"
  Sum2/1 -> positive half1/1  "HFL"
  Sum4/1 -> positive half4/1
  Divide10/1 -> Mux2/3  "SOL"
  positive half2/1 -> Mux1/2
  Divide14/1 -> Mux4/1  "HAM"
  theta_tgt [rad]/1 -> Sum1/1
  Demux5/5 -> Divide6/2  "SGainGLU_HAM"
  Divide6/1 -> positive half6/1  "HAM"
  positive half1/1 -> Mux1/1
  Mux1/1 -> E_M3 [HFL GLU HAM]/1
  Divide5/1 -> Sum8/2
  Demux8/3 -> Divide15/2  "LGainBFSH_VAS"
  parSt_M2/1 -> Demux8/1
  Demux8/1 -> Divide14/1  "FGain_HAM"
  Gain/1 -> Mux4/2  "VAS"
  Sum8/1 -> Divide6/1, positive half2/1  "GLU"
  Demux5/3 -> Divide4/2  "GainTh_GLU"
  Gain2/1 -> Divide19/1
  Divide20/1 -> Sum2/2
  Gain3/1 -> Divide20/1
  Divide19/1 -> Sum2/1
  parSt_M3/1 -> Demux5/1
  Divide4/1 -> Sum8/1
  Demux3/3 -> Divide10/1  "FGain_SOL"
  FmHAM/1 -> Divide14/2
  theta dtheta [rad rad/s]/1 -> Demux7/1
  Sum1/1 -> Gain2/1, Divide4/1
  Demux7/1 -> Sum1/2  "theta"
  Demux5/4 -> Divide5/2  "GainDTh_GLU"
  FmGAS/1 -> Divide11/2
  Demux8/4 -> Sum4/1  "loff_BFSH"
  FmVAS/1 -> Divide8/2
  Demux3/1 -> Divide7/1  "FGain_GLU"
  positive half4/1 -> Divide13/1
  Divide8/1 -> Mux2/2  "VAS"
  Demux3/2 -> Divide8/1  "FGain_VAS"
  Mux4/1 -> E_M2 [HAM VAS BFSH GAS]/1
  parStPreE/1 -> E_St_0/1
  Sum6/1 -> E_M5 [TA]/1  "TA"
  Demux1/5 -> Divide21/2  "SGainGLU_HAM"
  Divide12/1 -> Sum11/1
  Sum11/1 -> Mux5/2, Divide21/1  "GLU"
  Demux4/4 -> Divide9/2  "Exc_CRF"
  Divide21/1 -> Mux5/3  "HAM"
  CExc_HSw/1 -> Demux4/1
  Demux1/4 -> Divide9/1  "SGainCRF_GLU"
  Divide17/1 -> Sum7/2
  Demux1/2 -> Divide17/1  "SGainCHAM_HFL"
  Demux4/2 -> Divide22/2  "Exc_CGLU"
  Sum7/1 -> Mux5/1  "HFL"
  positive half5/1 -> Divide16/1
  Demux1/1 -> Divide22/1  "SGainCGLU_HFL"
  Demux4/1 -> Divide12/2  "Exc_CHFL"
  Demux4/3 -> Divide17/2  "Exc_CHAM"
  Divide9/1 -> Sum11/2
  Demux1/3 -> Divide12/1  "SGainCHFL_GLU"
  parSt_M4/1 -> Demux1/1
  Demux6/3 -> Divide25/2  "FGainSOL_TA"
  Demux6/1 -> Sum5/1  "loffTA"
  Demux6/2 -> Divide16/2  "LGain_TA"
  CtrlPar/1 -> parStPreE/1, parSt_M1/1, parSt_M2/1, parSt_M5/1, parSt_M4/1, parSt_M3/1
  Divide25/1 -> Sum6/2
  Mux5/1 -> E_M4 [HFL GLU HAM]/1
  Divide22/1 -> Sum7/1
  Sum5/1 -> positive half5/1
  Divide16/1 -> Sum6/1
  parSt_M5/1 -> Demux6/1
  FmSOL/1 -> Divide25/1, Divide10/2
  LceTA/1 -> Sum5/2

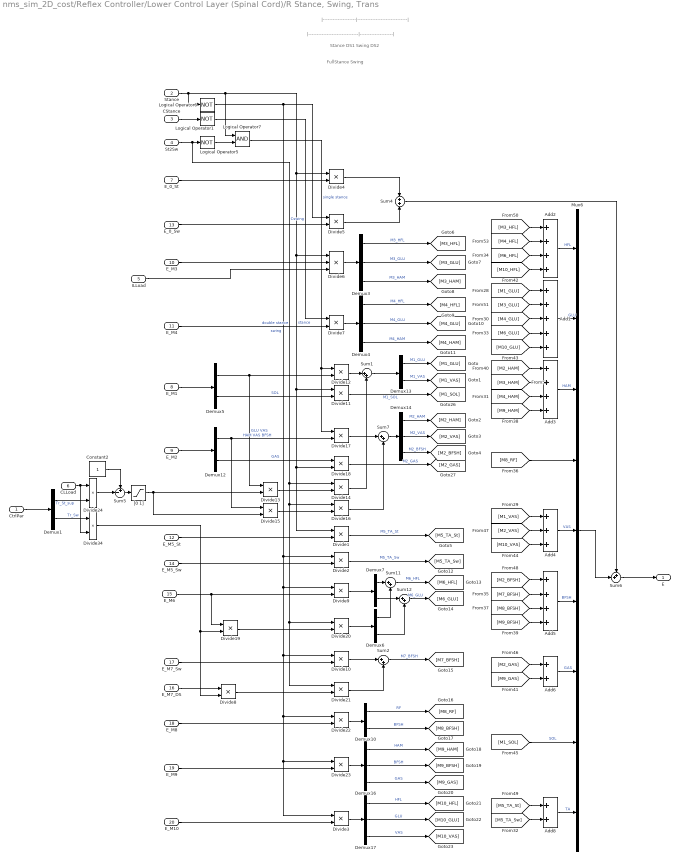
== system nms_sim_2D_cost/Reflex Controller/Lower Control Layer (Spinal Cord)/R Stance, Swing, Trans ==
  note: Stance DS1 Swing DS2
  note: FullStance Swing
  note: |------------------------------|--------------------|
  note: |--------------------|------------------------------|
  CtrlPar : Inport
  Stance : Inport  Port=2
  CStance : Inport  Port=3
  St2Sw : Inport  Port=4
  ILLoad : Inport  Port=5
  CLLoad : Inport  Port=6
  E_0_St : Inport  Port=7
  E_M1 : Inport  Port=8
  E_M2 : Inport  Port=9
  E_M3 : Inport  Port=10
  E_M4 : Inport  Port=11
  E_M5_St : Inport  Port=12
  E_0_Sw : Inport  Port=13
  E_M5_Sw : Inport  Port=14
  E_M6 : Inport  Port=15
  E_M7_DS : Inport  Port=16
  E_M7_Sw : Inport  Port=17
  E_M8 : Inport  Port=18
  E_M9 : Inport  Port=19
  E_M10 : Inport  Port=20
  Add1 : Sum  Inputs=5
  Add2 : Sum  Inputs=4
  Add3 : Sum  Inputs=4
  Add4 : Sum  Inputs=3
  Add5 : Sum  Inputs=4
  Add6 : Sum  Inputs=2
  Add8 : Sum  Inputs=2
  Constant2 : Constant
  Demux{1,6..7,10,13} (5 alike) : Demux  Outputs=2
  Demux12 : Demux  Outputs=[3 1]
  Demux{3..4,14,16..17} (5 alike) : Demux  Outputs=3
  Demux5 : Demux  Outputs=[2 1]
  Divide{1..5,7..24,34} (24 alike) : Product
  Divide6 : Product  Inputs=3
  Logical Operator1 : Logic  Operator=NOT  AllPortsSameDT=off  OutDataTypeStr=boolean
  Logical Operator5 : Logic  Operator=NOT  AllPortsSameDT=off  OutDataTypeStr=boolean
  Logical Operator6 : Logic  Operator=NOT  AllPortsSameDT=off  OutDataTypeStr=boolean
  Logical Operator7 : Logic  AllPortsSameDT=off  OutDataTypeStr=boolean
  Mux6 : Mux  Inputs=9
  Sum{1..2,7,11..12} (5 alike) : Sum  Inputs=|++  InputSameDT=on  SaturateOnIntegerOverflow=on  OutDataTypeStr=Inherit: Same as first input
  Sum4 : Sum  InputSameDT=on  SaturateOnIntegerOverflow=on  OutDataTypeStr=Inherit: Same as first input
  Sum5 : Sum  Inputs=+-|  InputSameDT=on  SaturateOnIntegerOverflow=on  OutDataTypeStr=Inherit: Same as first input
  Sum6 : Sum  Inputs=++|  InputSameDT=on  SaturateOnIntegerOverflow=on  OutDataTypeStr=Inherit: Same as first input
  "[0 1]" : Saturate  UpperLimit=1  LowerLimit=0  ZeroCross=off
  E : Outport  OutputWhenDisabled=reset  InitialOutput=0  VectorParamsAs1DForOutWhenUnconnected=off
  wires:
  CtrlPar/1 -> Demux1/1
  Stance/1 -> Logical Operator6/1, Logical Operator7/1, Divide4/1, Divide11/1, Divide18/2, Divide1/1, Divide6/1  "stance"
  St2Sw/1 -> Logical Operator5/1, Divide14/1, Divide16/1, Divide20/1, Divide21/1  "double stance"
  Logical Operator5/1 -> Logical Operator7/2
  E_M4/1 -> Divide7/2
  CStance/1 -> Logical Operator1/1
  Logical Operator1/1 -> Divide7/1  "Cswing"
  Demux1/1 -> Divide24/2  "Tr_St_sup"
  Divide24/1 -> Sum5/2
  Constant2/1 -> Sum5/1
  CLLoad/1 -> Divide24/1, Divide34/2
  Demux4/1 -> [M4_HFL]  "M4_HFL"
  Add2/1 -> Mux6/1  "HFL"
  Add1/1 -> Mux6/2  "GLU"
  Demux4/2 -> [M4_GLU]  "M4_GLU"
  Add3/1 -> Mux6/3  "HAM"
  Demux4/3 -> [M4_HAM]  "M4_HAM"
  Add4/1 -> Mux6/5  "VAS"
  Add5/1 -> Mux6/6  "BFSH"
  Add6/1 -> Mux6/7  "GAS"
  Add8/1 -> Mux6/9  "TA"
  Demux1/2 -> Divide34/1  "Tr_Sw"
  Divide7/1 -> Demux4/1
  Logical Operator7/1 -> Divide12/1, Divide17/1  "single stance"
  Divide34/1 -> Divide19/2, Divide8/2
  Logical Operator6/1 -> Divide5/1, Divide2/1, Divide9/1, Divide10/1, Divide23/1, Divide3/1, Divide22/1  "swing"
  Mux6/1 -> Sum6/2
  Sum6/1 -> E/1
  Sum4/1 -> Sum6/1
  E_0_Sw/1 -> Divide5/2
  E_0_St/1 -> Divide4/2
  Divide5/1 -> Sum4/2
  Divide4/1 -> Sum4/1
  E_M1/1 -> Demux5/1
  E_M2/1 -> Demux12/1
  Demux5/1 -> Divide12/2, Divide13/1  "GLU VAS"
  Demux5/2 -> Divide11/2  "SOL"
  Divide12/1 -> Sum1/1
  Divide13/1 -> Divide14/2
  Divide14/1 -> Sum1/2
  Divide16/1 -> Sum7/2
  Divide15/1 -> Divide16/2
  Sum1/1 -> Demux13/1
  Demux13/1 -> [M1_GLU]  "M1_GLU"
  Demux13/2 -> [M1_VAS]  "M1_VAS"
  Demux12/1 -> Divide17/2, Divide15/1  "HAM VAS BFSH"
  Divide17/1 -> Sum7/1
  Sum7/1 -> Demux14/1
  Demux14/1 -> [M2_HAM]  "M2_HAM"
  Demux14/2 -> [M2_VAS]  "M2_VAS"
  Demux14/3 -> [M2_BFSH]  "M2_BFSH"
  Demux12/2 -> Divide18/1  "GAS"
  Divide18/1 -> [M2_GAS]  "M2_GAS"
  E_M5_St/1 -> Divide1/2
  Divide1/1 -> [M5_TA_St]  "M5_TA_St"
  Divide11/1 -> [M1_SOL]  "M1_SOL"
  E_M3/1 -> Divide6/2
  ILLoad/1 -> Divide6/3
  Divide6/1 -> Demux3/1
  Demux3/1 -> [M3_HFL]  "M3_HFL"
  Demux3/2 -> [M3_GLU]  "M3_GLU"
  Demux3/3 -> [M3_HAM]  "M3_HAM"
  E_M5_Sw/1 -> Divide2/2
  Divide2/1 -> [M5_TA_Sw]  "M5_TA_Sw"
  E_M6/1 -> Divide9/2, Divide19/1
  Divide9/1 -> Demux7/1
  Demux7/2 -> Sum12/1
  Divide20/1 -> Demux6/1
  Demux6/1 -> Sum11/2
  Demux6/2 -> Sum12/2
  Demux7/1 -> Sum11/1
  Divide19/1 -> Divide20/2
  Sum11/1 -> [M6_HFL]  "M6_HFL"
  Sum12/1 -> [M6_GLU]  "M6_GLU"
  Divide10/1 -> Sum2/1
  Divide21/1 -> Sum2/2
  Sum5/1 -> "[0 1]"/1
  E_M7_Sw/1 -> Divide10/2
  Divide8/1 -> Divide21/2
  E_M7_DS/1 -> Divide8/1
  Sum2/1 -> [M7_BFSH]  "M7_BFSH"
  E_M8/1 -> Divide22/2
  Divide22/1 -> Demux10/1
  E_M9/1 -> Divide23/2
  Divide23/1 -> Demux16/1
  E_M10/1 -> Divide3/2
  Divide3/1 -> Demux17/1
  Demux10/2 -> [M8_BFSH]  "BFSH"
  Demux10/1 -> [M8_RF]  "RF"
  Demux16/1 -> [M9_HAM]  "HAM"
  Demux16/2 -> [M9_BFSH]  "BFSH"
  Demux16/3 -> [M9_GAS]  "GAS"
  Demux17/1 -> [M10_HFL]  "HFL"
  Demux17/2 -> [M10_GLU]  "GLU"
  Demux17/3 -> [M10_VAS]  "VAS"
  [M1_GLU] -> Add1/1
  [M3_GLU] -> Add1/2
  [M4_GLU] -> Add1/3
  [M6_GLU] -> Add1/4
  [M10_GLU] -> Add1/5
  [M1_VAS] -> Add4/1
  [M2_HAM] -> Add3/1
  [M2_VAS] -> Add4/2
  [M2_BFSH] -> Add5/1
  [M2_GAS] -> Add6/1
  [M3_HFL] -> Add2/1
  [M3_HAM] -> Add3/2
  [M4_HFL] -> Add2/2
  [M4_HAM] -> Add3/3
  [M5_TA_St] -> Add8/1
  [M5_TA_Sw] -> Add8/2
  [M6_HFL] -> Add2/3
  [M7_BFSH] -> Add5/2
  [M9_BFSH] -> Add5/4
  [M8_BFSH] -> Add5/3
  [M8_RF] -> Mux6/4
  [M9_HAM] -> Add3/4
  [M9_GAS] -> Add6/2
  [M10_HFL] -> Add2/4
  [M10_VAS] -> Add4/3
  [M1_SOL] -> Mux6/8  "SOL"
  "[0 1]"/1 -> Divide15/2, Divide13/2
